simulink model "Intermodal_simulation_IBonly_Dash"  (R2024b)
settings: Solver=VariableStepDiscrete  StartTime=0.0  StopTime=10000  RelTol=1e-3
model workspace (MAT data in the model file):
  HostlerTotal = Simulink.Parameter
  HostlerTotal.Value = 30
  HostlerTotal.Complexity = 'real'
  HostlerTotal.Dimensions = [1 1]
  HostlerTotal.DataType = 'auto'
  HostlerTotal.Min = 1
  HostlerTotal.Max = 50
  Train_interarrival = 179.78803498
  hostler_service_time = 20.171478921
  meanServiceTime = 25.1372997712
  num_entities = 30
undefined symbols (not defined in the file): m, n
settings Model: SimulationMode=accelerator  PacingRate=112  Creator=calskiles  LastModifiedBy=imagined
settings SolverCC: MinimalZcImpactIntegration=on
settings DataIOCC: SaveFormat=StructureWithTime
settings DebuggingCC: ReadBeforeWriteMsg=DisableAll  WriteAfterWriteMsg=DisableAll  WriteAfterReadMsg=DisableAll  MultiTaskDSMMsg=none
settings ModelReferenceCC: UpdateModelReferenceTargets=IfOutOfDate
settings SFSimCC: SFSimEcho=off
settings ConfigComp: CovEnable=on  RecordCoverage=on  CovNameIncrementing=on  CovSaveSingleToWorkspaceVar=on  CovModelRefEnable=on

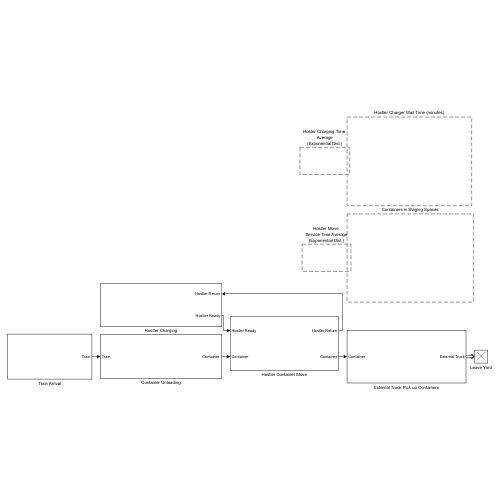
[thumbnail: Simulink's stored preview of the top-level diagram]
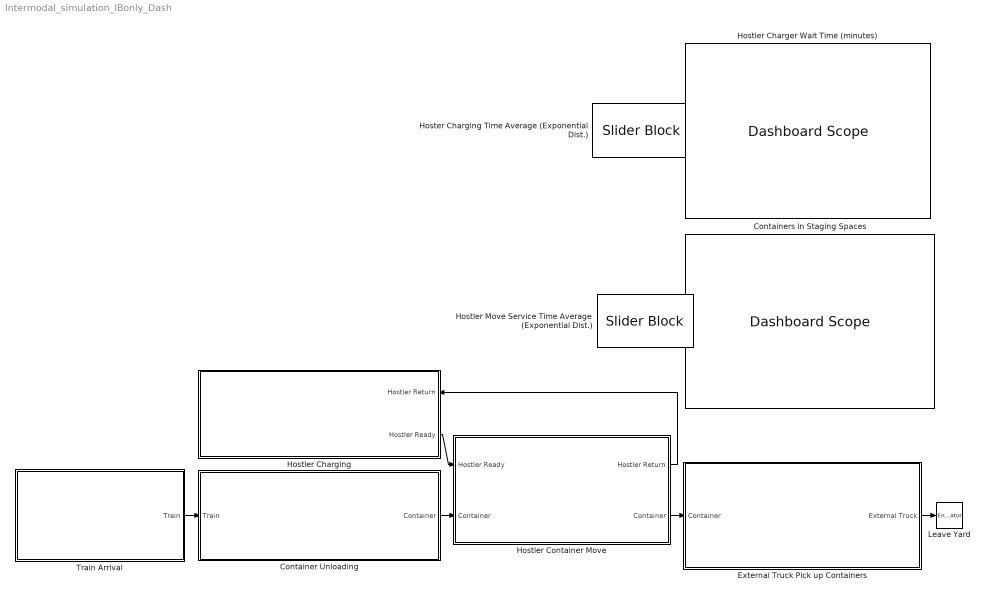
== system Intermodal_simulation_IBonly_Dash ==
  Container Unloading : Subsystem
  Containers in Staging Spaces : DashboardScope  Ymin=0  Ymax=300  ScaleAtStop=off
  External Truck Pick up Containers : Subsystem
  Hoster Charging Time Average (Exponential Dist.) : SliderBlock  ScaleMax=90  TickInterval=15
  Hostler Charger Wait Time (minutes) : DashboardScope  Ymin=0  Ymax=100  ScaleAtStop=off
  Hostler Charging : Subsystem
      settings: PortSchema="{\"entries\":[{\"content\":{\"sides\":[{\"content\":{},\"type\":\"ConnectorPlacement.EquallySpacedRectSide\",\"uuid\":\"3ce774db-239e-416c-9591-362e2bcf1a2e\"},{\"content\":{\"connectorIds\":[\"In1\",\"Out1\"],\"side\":\"RIGHT\"},\"type\":\"ConnectorPlacement.EquallySpacedRectSide\",\"uuid\":\"4f8c07a4-3f87-4675-89ca-af788f15d8e0\"},{\"content\":{\"side\":\"TOP\"},\"type\":\"ConnectorPlacement.EquallySpacedRectSide\",\"uuid\":\"72da7e6e-2bc7-41b8-bd1a-18f8b2245bef\"}]},\"type\":\"ConnectorPlacement.EquallySpacedConnector\",\"uuid\":\"ba1be72f-2972-46a9-ae69-d157b6b82304\"}],\"packageUris\":[\"http://schema.mathworks.com/mf0/Connector/R2020b\"],\"version\":\"1.0\"}"
  Hostler Container Move : Subsystem
  Hostler Move Service Time Average (Exponential Dist.) : SliderBlock  ScaleMin=5  ScaleMax=45  TickInterval=10
  Leave Yard : EntityTerminator  InputPortMessageModes=m
  Train Arrival : Subsystem
  wires:
  Train Arrival/1(Train) -> Container Unloading/1(Train)
  External Truck Pick up Containers/1(External Truck) -> Leave Yard/1
  Hostler Charging/1(Hostler Ready) -> Hostler Container Move/1(Hostler Ready)
  Container Unloading/1("Container ") -> Hostler Container Move/2("Container ")
  Hostler Container Move/1(Hostler Return) -> Hostler Charging/1(Hostler Return)
  Hostler Container Move/2(Container) -> External Truck Pick up Containers/1(Container)

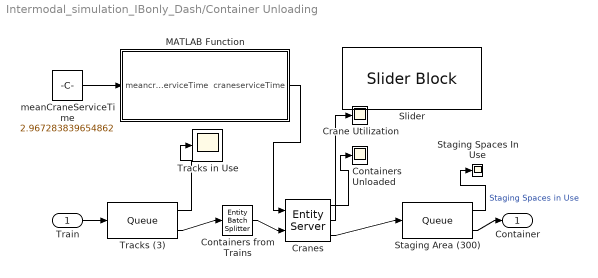
== system Intermodal_simulation_IBonly_Dash/Container Unloading ==
  Train : Inport
  Containers Unloaded : Scope
  Containers from Trains : EntityBatchSplitter  InputPortMessageModes=m  OutputPortMessageModes=m
      settings: OutputPortMap=o4
  Crane Utilization : Scope
  Cranes : EntityServer  InputPortMessageModes=n,m  OutputPortMessageModes=n,n,m  ServiceTimeSource=Signal port  ServiceTimeValue=3  NumberEntitiesDeparted=on  Utilization=on
      settings: InputPortMap=u0,u2  OutputPortMap=o0,o5,o9
  MATLAB Function : MATLAB Function  TreatAsAtomicUnit=on
  Slider : SliderBlock  ScaleMin=1  ScaleMax=10  TickInterval=1
  Staging Area (300) : Queue  InputPortMessageModes=m  OutputPortMessageModes=n,m  Capacity=300  AverageQueueLength=on
      settings: OutputPortMap=o3,o5
  Staging Spaces In Use : Scope
  Tracks (3) : Queue  InputPortMessageModes=m  OutputPortMessageModes=n,m  Capacity=3  NumberEntitiesInBlock=on
      settings: OutputPortMap=o1,o5
  Tracks in Use : Scope
  meanCraneServiceTime : Constant  Value=2.967283839654862
  "Container " : Outport
  wires:
  Staging Area (300)/2 -> "Container "/1
  Containers from Trains/1 -> Cranes/2
  Tracks (3)/2 -> Containers from Trains/1
  Tracks (3)/1 -> Tracks in Use/1
  Staging Area (300)/1 -> Staging Spaces In Use/1  "Staging Spaces in Use"
  Cranes/3 -> Staging Area (300)/1
  Cranes/1 -> Containers Unloaded/1
  Train/1 -> Tracks (3)/1
  Cranes/2 -> Crane Utilization/1
  MATLAB Function/1(craneserviceTime) -> Cranes/1
  meanCraneServiceTime/1 -> MATLAB Function/1(meancraneServiceTime)

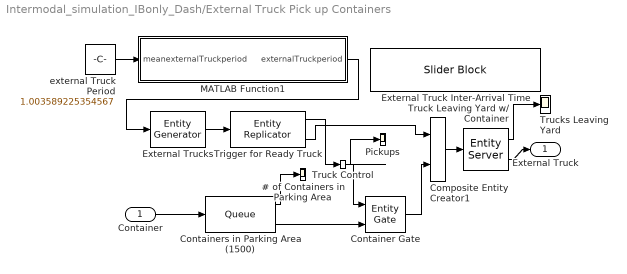
== system Intermodal_simulation_IBonly_Dash/External Truck Pick up Containers ==
  Container : Inport
  " Truck Leaving Yard w/ Container" : EntityServer  InputPortMessageModes=m  OutputPortMessageModes=n,m  Capacity=2  ServiceTimeValue=.5  NumberEntitiesDeparted=on
      settings: OutputPortMap=o0,o9
  # of Containers in Parking Area : Scope
  Composite Entity Creator1 : CompositeEntityCreator  InputPortMessageModes=m,m  OutputPortMessageModes=m  EntityTypeName=Combined_external
      settings: InputPortMap=u0,u1
  Container Gate : EntityGate  InputPortMessageModes=m,m  OutputPortMessageModes=m  OperatingMode=Release gate
  Containers in Parking Area (1500) : Queue  InputPortMessageModes=m  OutputPortMessageModes=n,m  Capacity=5000  NumberEntitiesInBlock=on
      settings: OutputPortMap=o1,o5
  External Truck Inter-Arrival Time : SliderBlock  ScaleMax=10  TickInterval=1
  External Trucks : EntityGenerator  OutputPortMessageModes=m  TimeSource=Signal port  Period=3  EntityType=Structured  EntityTypeName=Entity
      settings: InputPortMap=u1
  MATLAB Function1 : MATLAB Function  TreatAsAtomicUnit=on
  Pickups : Scope
  Trigger for Ready Truck : EntityReplicator  InputPortMessageModes=m  OutputPortMessageModes=m,m  HoldOriginalEntityUntilAllReplicasDepart=on
  Truck Control : EntityGenerator  InputPortMessageModes=m  OutputPortMessageModes=n,m  GenerationMethod=Event-based  AttributeName=entity  AttributeInitialValue=0  NumberEntitiesDeparted=on  EntityTypeName=Entity
      settings: InputPortMap=u0  OutputPortMap=o0,o3
  Trucks Leaving Yard : Scope
  external Truck Period : Constant  Value=1.003589225354567
  External Truck : Outport
  wires:
  Container/1 -> Containers in Parking Area (1500)/1
  " Truck Leaving Yard w/ Container"/2 -> External Truck/1
  Composite Entity Creator1/1 -> " Truck Leaving Yard w/ Container"/1
  Containers in Parking Area (1500)/2 -> Container Gate/2
  " Truck Leaving Yard w/ Container"/1 -> Trucks Leaving Yard/1
  Trigger for Ready Truck/2 -> Composite Entity Creator1/1
  Container Gate/1 -> Composite Entity Creator1/2
  Truck Control/2 -> Container Gate/1
  Trigger for Ready Truck/1 -> Truck Control/1
  Truck Control/1 -> Pickups/1
  External Trucks/1 -> Trigger for Ready Truck/1
  Containers in Parking Area (1500)/1 -> # of Containers in Parking Area/1
  MATLAB Function1/1(externalTruckperiod) -> External Trucks/1
  external Truck Period/1 -> MATLAB Function1/1(meanexternalTruckperiod)

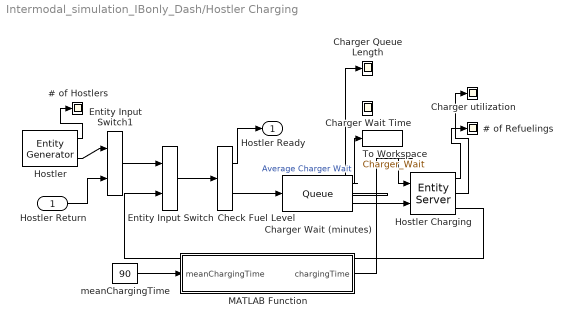
== system Intermodal_simulation_IBonly_Dash/Hostler Charging ==
  Hostler Return : Inport
  # of Hostlers : Scope
  # of Refuelings : Scope
  Charger Queue Length : Scope
  Charger Wait (minutes) : Queue  InputPortMessageModes=m  OutputPortMessageModes=n,n,m  Capacity=20  AverageWait=on  AverageQueueLength=on
      settings: OutputPortMap=o2,o3,o5
  Charger Wait Time : Scope
  Charger utilization : Scope
  Check Fuel Level : EntityOutputSwitch  InputPortMessageModes=m  OutputPortMessageModes=m,m  SwitchingCriterion=From attribute  SwitchAttributeName=fuel_level
  Entity Input Switch : EntityInputSwitch  InputPortMessageModes=m,m  OutputPortMessageModes=m
  Entity Input Switch1 : EntityInputSwitch  InputPortMessageModes=m,m  OutputPortMessageModes=m
  Hostler : EntityGenerator  OutputPortMessageModes=n,m  TimeSource=MATLAB action  Period=0  IntergenerationTimeAction=|  GenerateEntityAtSimulationStart=off  AttributeName=fuel_level  NumberEntitiesDeparted=on  EntityType=Structured  EntityTypeName=Hostler
      | persistent count igt num_entities;
      | 
      | % Initialize count and igt on the first call
      | if isempty(count)
      |     % User-defined input for number of entities
      |     num_entities = 30; % Change this to a user input or pass it as a parameter
      | 
      |     % Create the intergeneration time array for the given number of entities
      |     igt = [zeros(1, num_entities) inf]; % Generate 'num_entities' entities, then stop
      | 
      |     count = 0; % Start count at 0 to ensure correct number of entities
      | end
      | 
      | % Increment count for the next entity generation
      | count = count + 1;
      | 
      | % Set intergeneration time (dt) for the current entity
      | dt = igt(count);
      | 
      | % Stop after generating the desired number of entities
      | if count > num_entities
      |     dt = inf; % Prevent further entity generation
      | end
      settings: OutputPortMap=o0,o3
  Hostler Charging : EntityServer  InputPortMessageModes=n,m  OutputPortMessageModes=n,n,m  Capacity=8  ServiceTimeSource=Signal port  ServiceTimeValue=44.9126226067589  ServiceCompleteAction=entity.fuel_level = 1;  NumberEntitiesDeparted=on  Utilization=on
      settings: InputPortMap=u0,u2  OutputPortMap=o0,o5,o9
  MATLAB Function : MATLAB Function  TreatAsAtomicUnit=on
  To Workspace : ToWorkspace  VariableName=Charger_Wait  SaveFormat=Structure With Time  SampleTime=-1
  meanChargingTime : Constant  Value=90
  Hostler Ready : Outport
  wires:
  Hostler/1 -> # of Hostlers/1
  Charger Wait (minutes)/3 -> Hostler Charging/2
  Check Fuel Level/1 -> Hostler Ready/1
  Hostler/2 -> Entity Input Switch1/1
  Hostler Return/1 -> Entity Input Switch1/2
  Check Fuel Level/2 -> Charger Wait (minutes)/1
  Hostler Charging/3 -> Entity Input Switch/2
  Entity Input Switch1/1 -> Entity Input Switch/1
  Entity Input Switch/1 -> Check Fuel Level/1
  Hostler Charging/2 -> Charger utilization/1
  Charger Wait (minutes)/2 -> Charger Queue Length/1
  Hostler Charging/1 -> # of Refuelings/1
  MATLAB Function/1(chargingTime) -> Hostler Charging/1
  meanChargingTime/1 -> MATLAB Function/1(meanChargingTime)
  Charger Wait (minutes)/1 -> To Workspace/1  "Average Charger Wait"

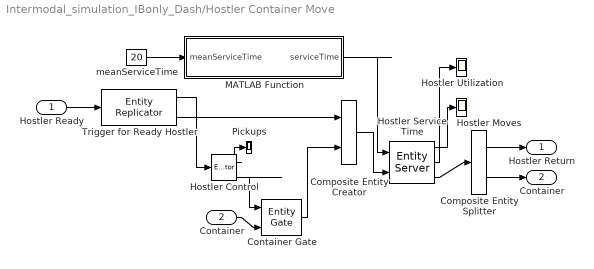
== system Intermodal_simulation_IBonly_Dash/Hostler Container Move ==
  Hostler Ready : Inport
  "Container " : Inport  Port=2
  Composite Entity Creator : CompositeEntityCreator  InputPortMessageModes=m,m  OutputPortMessageModes=m  EntityTypeName=Combined
      settings: InputPortMap=u0,u1
  Composite Entity Splitter : CompositeEntitySplitter  InputPortMessageModes=m  OutputPortMessageModes=m,m
      settings: OutputPortMap=o0,o1
  Container Gate : EntityGate  InputPortMessageModes=m,m  OutputPortMessageModes=m  OperatingMode=Release gate
  Hostler Control : EntityGenerator  InputPortMessageModes=m  OutputPortMessageModes=n,m  GenerationMethod=Event-based  AttributeName=entity  AttributeInitialValue=0  NumberEntitiesDeparted=on  EntityTypeName=Entity
      settings: InputPortMap=u0  OutputPortMap=o0,o3
  Hostler Moves : Scope
  Hostler Service Time : EntityServer  InputPortMessageModes=n,m  OutputPortMessageModes=n,n,m  Capacity=num_entities  ServiceTimeSource=Signal port  ServiceTimeValue=10  ServiceTimeAction=dt = rand(10,20);  ServiceCompleteAction=entity.E1.fuel_level = entity.E1.fuel_level + hostler_service_time*.0035;  NumberEntitiesDeparted=on  Utilization=on
      settings: InputPortMap=u0,u2  OutputPortMap=o0,o5,o9
  Hostler Utilization : Scope
  MATLAB Function : MATLAB Function  TreatAsAtomicUnit=on
  Pickups : Scope
  Trigger for Ready Hostler : EntityReplicator  InputPortMessageModes=m  OutputPortMessageModes=m,m  HoldOriginalEntityUntilAllReplicasDepart=on
  meanServiceTime : Constant  Value=20
  Hostler Return : Outport
  Container : Outport  Port=2
  wires:
  Composite Entity Splitter/1 -> Hostler Return/1
  Hostler Service Time/2 -> Hostler Utilization/1
  Hostler Service Time/3 -> Composite Entity Splitter/1
  Composite Entity Creator/1 -> Hostler Service Time/2
  Composite Entity Splitter/2 -> Container/1
  "Container "/1 -> Container Gate/2
  Container Gate/1 -> Composite Entity Creator/2
  Hostler Ready/1 -> Trigger for Ready Hostler/1
  Trigger for Ready Hostler/2 -> Composite Entity Creator/1
  Hostler Control/2 -> Container Gate/1
  Trigger for Ready Hostler/1 -> Hostler Control/1
  Hostler Service Time/1 -> Hostler Moves/1
  Hostler Control/1 -> Pickups/1
  MATLAB Function/1(serviceTime) -> Hostler Service Time/1
  meanServiceTime/1 -> MATLAB Function/1(meanServiceTime)

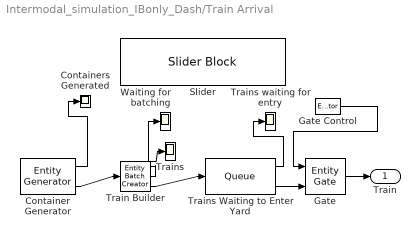
== system Intermodal_simulation_IBonly_Dash/Train Arrival ==
  Container Generator : EntityGenerator  OutputPortMessageModes=n,m  AttributeName=Size  NumberEntitiesDeparted=on  EntityType=Structured  EntityTypeName=Containers
      settings: OutputPortMap=o0,o3
  Containers Generated : Scope
  Gate : EntityGate  InputPortMessageModes=m,m  OutputPortMessageModes=m  OperatingMode=Release gate  OpenGateAtSimulationStart=on
  Gate Control : EntityGenerator  OutputPortMessageModes=m  Period=Train_interarrival  AttributeName=entity  AttributeInitialValue=0  EntityTypeName=Entity
  Slider : SliderBlock  ScaleMin=60  ScaleMax=240
  Train Builder : EntityBatchCreator  InputPortMessageModes=m  OutputPortMessageModes=n,n,m  NumberOfEntitiesInBatch=300  EntityTypeName=Train  InputEntityName=Container  NumberOfEntitiesDeparted=on  NumberOfEntitiesRequiredForNextBatch=on
      settings: OutputPortMap=o1,o2,o4
  Trains : Scope
  Trains Waiting to Enter Yard : Queue  InputPortMessageModes=m  OutputPortMessageModes=n,m  Capacity=100  NumberEntitiesInBlock=on
      settings: OutputPortMap=o1,o5
  Trains waiting for entry : Scope
  Waiting for batching : Scope
  Train : Outport
  wires:
  Container Generator/2 -> Train Builder/1
  Train Builder/1 -> Trains/1
  Gate Control/1 -> Gate/1
  Container Generator/1 -> Containers Generated/1
  Train Builder/2 -> Waiting for batching/1
  Trains Waiting to Enter Yard/1 -> Trains waiting for entry/1
  Train Builder/3 -> Trains Waiting to Enter Yard/1
  Trains Waiting to Enter Yard/2 -> Gate/2
  Gate/1 -> Train/1

== matlab function Intermodal_simulation_IBonly_Dash/Hostler Container Move/MATLAB Function ==
  data: meanServiceTime input; serviceTime output
function serviceTime = computeServiceTime(meanServiceTime)
    % Generate service time using an exponential distribution
    serviceTime = exprnd(meanServiceTime);
    hostler_service_time = serviceTime;
end

== matlab function Intermodal_simulation_IBonly_Dash/External Truck Pick up Containers/MATLAB Function1 ==
  data: meanexternalTruckperiod input; externalTruckperiod output
function externalTruckperiod = computeexternalTruckperiod(meanexternalTruckperiod)
   % Generate service time based on the exponential distribution
   externalTruckperiod = exprnd(meanexternalTruckperiod);
end

== matlab function Intermodal_simulation_IBonly_Dash/Container Unloading/MATLAB Function ==
  data: meancraneServiceTime input; craneserviceTime output
function craneserviceTime = computeServiceTime(meancraneServiceTime)
    % Generate service time using an exponential distribution
    craneserviceTime = exprnd(meancraneServiceTime);
end

== matlab function Intermodal_simulation_IBonly_Dash/Hostler Charging/MATLAB Function ==
  data: meanChargingTime input; chargingTime output
function chargingTime = computeChargingTime(meanChargingTime)
   % Generate service time based on the exponential distribution
   chargingTime = exprnd(meanChargingTime);
end
